simulink model "furuta_single_inverted_pendulum_model_CL"  (R2025a)
settings: Solver=ode4  StartTime=0.0  StopTime=inf  FixedStep=0.0001  RelTol=1e-3
InitFcn:
  | addpath('functions');
model workspace (MATLAB code in the model file):
  | arm_torque = 0;
  | L_arm = 0.2;
  | I_arm = 0.01;
  | lcom_1 = 0.6;
  | I_1 = 0.02;
  | m_1 = 1;
  | L_1 = 1;
  | 
  | init_cond = [pi/2; 0; 0.01; 0];
settings Model: Creator=Esther  LastModifiedBy=marcus

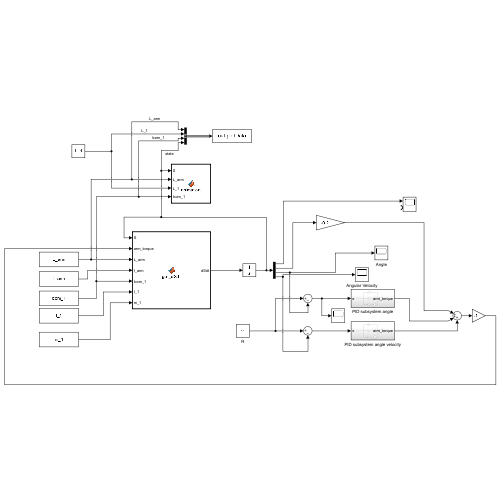
[thumbnail: Simulink's stored preview of the top-level diagram]
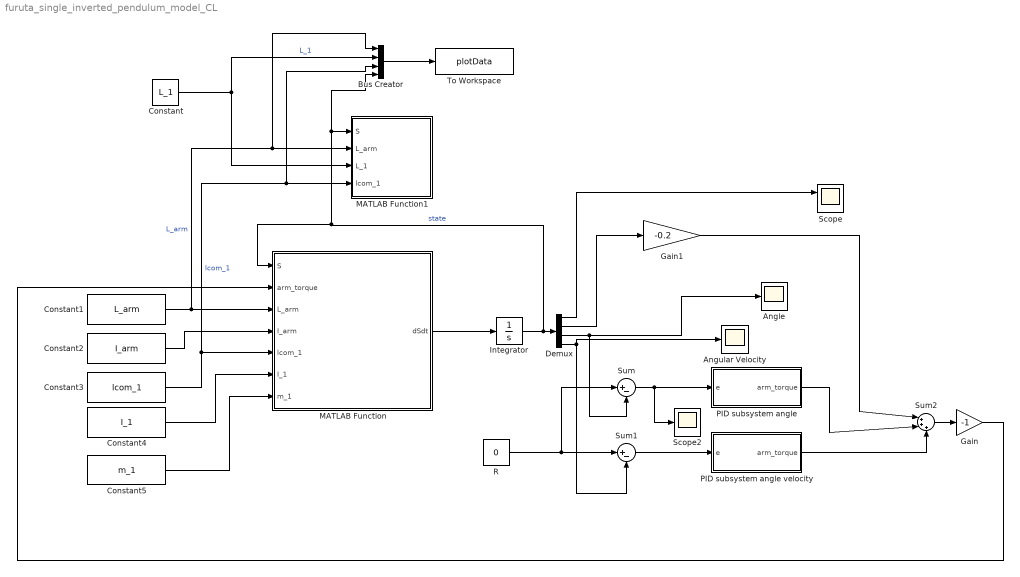
== system furuta_single_inverted_pendulum_model_CL ==
  Angle : Scope
      settings: ActiveDisplayYMinimum=-6.9679733150236753  ActiveDisplayYMaximum=4.0512303756780108
  Angular Velocity : Scope
      settings: ActiveDisplayYMinimum=-3875.8658390527003  ActiveDisplayYMaximum=3642.7464695660938  DataLoggingVariableName=ScopeData2
  Bus Creator : BusCreator  Inputs=4
  Constant : Constant  Value=L_1
  Constant1 : Constant  Value=L_arm
  Constant2 : Constant  Value=I_arm
  Constant3 : Constant  Value=lcom_1
  Constant4 : Constant  Value=I_1
  Constant5 : Constant  Value=m_1
  Demux : Demux
  Gain : Gain  Gain=-1
  Gain1 : Gain  Gain=-0.2
  Integrator : Integrator  InitialCondition=init_cond
  MATLAB Function : MATLAB Function  TreatAsAtomicUnit=on
  MATLAB Function1 : MATLAB Function  TreatAsAtomicUnit=on
  PID subsystem angle : Subsystem
  PID subsystem angle velocity : Subsystem
  R : Constant  Value=0
  Scope : Scope  NumInputPorts=2
      settings: ActiveDisplayYMinimum=-1  ActiveDisplayYMaximum=1
  Scope2 : Scope
      settings: ActiveDisplayYMinimum=-2.6212708840748387  ActiveDisplayYMaximum=0.28014120934164871  DataLoggingVariableName=ScopeData4
  Sum : Sum  Inputs=|+-
  Sum1 : Sum  Inputs=|+-
  Sum2 : Sum  Inputs=|+++
  To Workspace : ToWorkspace  VariableName=plotData  SaveFormat=Timeseries  SampleTime=-1
  wires:
  MATLAB Function/1(dSdt) -> Integrator/1
  Constant1/1 -> MATLAB Function/3(L_arm), Bus Creator/1, MATLAB Function1/2(L_arm)  "L_arm"
  Constant2/1 -> MATLAB Function/4(I_arm)
  Constant3/1 -> Bus Creator/3, MATLAB Function1/4(lcom_1), MATLAB Function/5(lcom_1)  "lcom_1"
  Constant4/1 -> MATLAB Function/6(I_1)
  Constant5/1 -> MATLAB Function/7(m_1)
  Integrator/1 -> MATLAB Function/1(S), MATLAB Function1/1(S), Bus Creator/4, Demux/1  "state"
  Bus Creator/1 -> To Workspace/1
  Constant/1 -> Bus Creator/2, MATLAB Function1/3(L_1)  "L_1"
  Demux/1 -> Scope/1
  R/1 -> Sum1/1, Sum/1
  Demux/3 -> Angle/1, Sum/2
  Demux/4 -> Angular Velocity/1, Sum1/2
  Sum/1 -> Scope2/1, PID subsystem angle/1(e)
  Sum1/1 -> PID subsystem angle velocity/1(e)
  Sum2/1 -> Gain/1
  Gain/1 -> MATLAB Function/2(arm_torque)
  Demux/2 -> Gain1/1
  Gain1/1 -> Sum2/1
  PID subsystem angle/1(arm_torque) -> Sum2/2
  PID subsystem angle velocity/1(arm_torque) -> Sum2/3

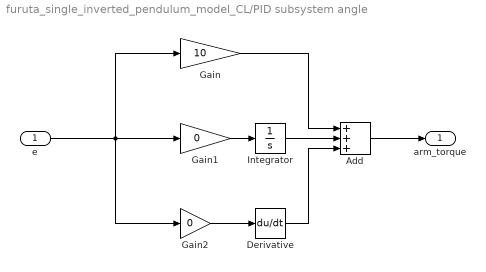
== system furuta_single_inverted_pendulum_model_CL/PID subsystem angle ==
  e : Inport
  Add : Sum  Inputs=+++
  Derivative : Derivative
  Gain : Gain  Gain=10
  Gain1 : Gain  Gain=0
  Gain2 : Gain  Gain=0
  Integrator : Integrator
  arm_torque : Outport
  wires:
  e/1 -> Gain2/1, Gain/1, Gain1/1
  Gain1/1 -> Integrator/1
  Gain2/1 -> Derivative/1
  Gain/1 -> Add/1
  Integrator/1 -> Add/2
  Derivative/1 -> Add/3
  Add/1 -> arm_torque/1

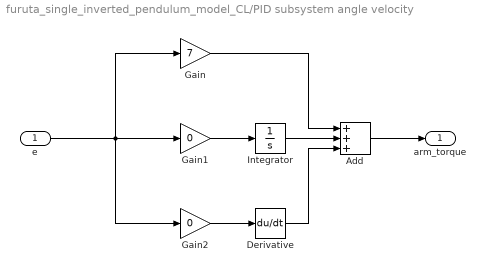
== system furuta_single_inverted_pendulum_model_CL/PID subsystem angle velocity ==
  e : Inport
  Add : Sum  Inputs=+++
  Derivative : Derivative
  Gain : Gain  Gain=7
  Gain1 : Gain  Gain=0
  Gain2 : Gain  Gain=0
  Integrator : Integrator
  arm_torque : Outport
  wires:
  e/1 -> Gain2/1, Gain/1, Gain1/1
  Gain1/1 -> Integrator/1
  Gain2/1 -> Derivative/1
  Gain/1 -> Add/1
  Integrator/1 -> Add/2
  Derivative/1 -> Add/3
  Add/1 -> arm_torque/1

== matlab function furuta_single_inverted_pendulum_model_CL/MATLAB Function1 ==
  settings: updateMethod=DISCRETE
  data: S input; L_arm input; L_1 input; lcom_1 input
function animation(S, L_arm, L_1, lcom_1)
    update_ratio = 100;
    realtime_animation_single(S, L_arm, L_1, lcom_1, update_ratio);
end

== matlab function furuta_single_inverted_pendulum_model_CL/MATLAB Function ==
  data: S input size=4; dSdt output size=4; arm_torque input size=1; L_arm input size=1; I_arm input size=1; lcom_1 input size=1; I_1 input size=1; m_1 input size=1
function dSdt = get_dSdt(S, arm_torque, L_arm, I_arm, lcom_1, I_1, m_1)
    t = 0;
    g = 9.81;
    phys_param = [L_arm, I_arm, lcom_1, I_1, m_1, g];
    fric_arm = [0.018, 0.018, 100];
    fric_1 = [0.0001, 0.0001, 100];
    dSdt = furuta_single_state_derivative(t, S, arm_torque, phys_param, fric_arm, fric_1);
end
